simulink model "homeMobileManipulator"  (R2026a)
settings: Solver=ode4  StartTime=0  StopTime=Inf  FixedStep=cfg.rates.plant  MaxStep=cfg.rates.plant  AbsTol=1e-8
PostLoadFcn:
  | hmmSetup;
InitFcn:
  | hmmInitializeRun(bdroot);
values from neighbouring files (symbols this model uses):
  armJointLimits = zeros(numel(idx.arm), 2)    [hmmSetup.m]
  cfg = app.RunCfg    [HomeMobileManipulatorApp.m]    (also in HomeMobileManipulatorExample.m = params.cfg; hmmSetup.m = hmmConfig(); setupParams.m = data.cfg)
undefined symbols (not defined in the file or in its folder): actionQueueInit, actorNameTable, Angle, apertureMap, armPlanInit, Axis, basePlanInit, Custom, Extent, gray, gripperCoupling, invalidRayHits, movableRegistry, objectTargetInit, perceptionStatusInit, placeTargetInit, Position, robotStateInit, Sim3dSensor
libraries: robotmaniplib x20, robotcorelib x18, simulink x9, sim3dcameralib x6, sim3dgroundtruthsensorlib x4, dspmtrx3 x3, slpidlib x3, sim3dlib x3, hdlsllib x2, robotsim3dlib x1
(part 4 of 6)

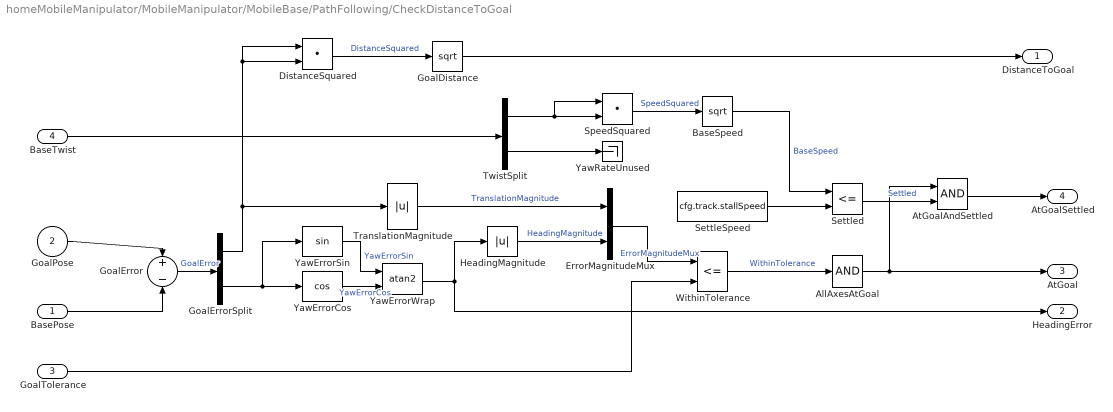
== system homeMobileManipulator/MobileManipulator/MobileBase/PathFollowing/CheckDistanceToGoal ==
  BasePose : Inport
  GoalPose : Inport  Port=2
  GoalTolerance : Inport  Port=3
  BaseTwist : Inport  Port=4
  AllAxesAtGoal : Logic  Inputs=1  IconShape=distinctive  AllPortsSameDT=off  OutDataTypeStr=boolean
  AtGoalAndSettled : Logic  Description=|  AllPortsSameDT=off  OutDataTypeStr=boolean
      | THE SUPERVISOR'S ARRIVAL TEST, WHICH IS NOT THE SAME SIGNAL THAT STOPS THE BASE.
      | 
      | AllAxesAtGoal alone is a POSITION test. Measured on the 40 s run of 2026-09-30 the
      | place leg reported HOLDING/DONE at t = 15.19 s while the chassis was still doing
      | 0.383 m/s, and the base then rolled a further 67.9 mm down its acceleration limit
      | (1.08 m/s^2, so 0.383^2/(2*1.08) = 67.9 mm - the ramp accounts for all of it). That is
      | more travel than the 80 mm per axis the goal was specified to, and it happens while the
      | arm is already planning: ArmSupervisor requested its place plan at 15.22 s, so the plan
      | was built on a base pose 64 mm stale.
      | 
      | cfg.track.goalHoldTime = 0.20 s does not catch this. It is a dwell on POSITION, and at
      | 0.4 m/s the chassis crosses 80 mm during the dwell, so the dwell is satisfied at cruise.
      | 
      | WHY THIS IS A SECOND SIGNAL AND NOT AN EXTRA TERM ON AtGoal. ZeroVelocityAtGoal in the
      | parent takes the RAW AllAxesAtGoal output and that is what commands zero velocity. AND
      | the settle term into that same signal and the command is never zeroed, so the base never
      | settles, so the term never becomes true - a deadlock. The raw test therefore stays on the
      | switch and only the signal leaving for BaseSupervisor carries the settle term. Because the
      | command is already zero by then, the plant decelerates at its own limit and this output is
      | guaranteed to go true within v/a, about 0.36 s on the measured run.
      | 
      | SAFE AGAINST THE STALL DETECTOR. BaseSupervisor/Following accumulates tProgress whenever
      | DistanceToGoal fails to improve by dProgressMin and declares Stalled at cfg.track.stallTime
      | = 2.00 s. Reconstructed from the same run, tProgress was 0.160 s at the arrival flip, so
      | there is 1.84 s of spare against the 0.36 s this adds.
      | 
      | TRANSLATION ONLY, DELIBERATELY. cfg.track.stallSpeed is in m/s. A yaw-rate term would need
      | a constant the configuration does not have, and the measured overshoot was pure translation
      | - vy and omega were both exactly zero from t = 15.08 s. Inventing a rate bound to cover a
      | case nothing has measured would be a worse trade than recording the limit here.
  BaseSpeed : Sqrt
  DistanceSquared : DotProduct  OutDataTypeStr=Inherit: Inherit via internal rule
  ErrorMagnitudeMux : Mux  Inputs=2
  GoalDistance : Sqrt
  GoalError : Sum  Inputs=+-
  GoalErrorSplit : Demux  Outputs=[2 1]
  HeadingMagnitude : Abs  SaturateOnIntegerOverflow=off
  SettleSpeed : Constant  Description=|  Value=cfg.track.stallSpeed
      | The speed below which the chassis counts as stopped. This is cfg.track.stallSpeed, the
      | same constant the stall detector already uses for "no progress", rather than a new one:
      | 0.020 m/s is either a speed worth noticing or it is not, and it cannot be both.
      | 
      | At this threshold the roll left after arrival is 0.020^2/(2*1.08) = 0.19 mm, against
      | 67.9 mm before the settle term existed.
  Settled : RelationalOperator  Operator=<=  OutDataTypeStr=boolean  RndMeth=Simplest  InputSameDT=off
  SpeedSquared : DotProduct  OutDataTypeStr=Inherit: Inherit via internal rule
  TranslationMagnitude : Abs  SaturateOnIntegerOverflow=off
  TwistSplit : Demux  Description=|  Outputs=[2 1]
      | BaseTwist is the REALISED body-frame [vx vy omega] after wheel saturation, not the
      | command - which is the whole point, since the command is already zero while the chassis
      | is still rolling. Split [2 1] so the translational pair can be normed on its own; the
      | yaw rate is deliberately not used, see AtGoalAndSettled.
  WithinTolerance : RelationalOperator  Operator=<=  OutDataTypeStr=boolean  RndMeth=Simplest  InputSameDT=off
  YawErrorCos : Trigonometry  Operator=cos
  YawErrorSin : Trigonometry
  YawErrorWrap : Trigonometry  Operator=atan2
  YawRateUnused : Terminator
  DistanceToGoal : Outport
  HeadingError : Outport  Port=2
  AtGoal : Outport  Port=3
  AtGoalSettled : Outport  Port=4
  wires:
  AtGoalAndSettled/1 -> AtGoalSettled/1
  Settled/1 -> AtGoalAndSettled/2  "Settled"
  SettleSpeed/1 -> Settled/2
  BaseSpeed/1 -> Settled/1  "BaseSpeed"
  GoalTolerance/1 -> WithinTolerance/2
  SpeedSquared/1 -> BaseSpeed/1  "SpeedSquared"
  HeadingMagnitude/1 -> ErrorMagnitudeMux/2  "HeadingMagnitude"
  TwistSplit/2 -> YawRateUnused/1
  YawErrorWrap/1 -> HeadingMagnitude/1, HeadingError/1
  AllAxesAtGoal/1 -> AtGoal/1, AtGoalAndSettled/1
  TranslationMagnitude/1 -> ErrorMagnitudeMux/1  "TranslationMagnitude"
  ErrorMagnitudeMux/1 -> WithinTolerance/1  "ErrorMagnitudeMux"
  BaseTwist/1 -> TwistSplit/1
  GoalDistance/1 -> DistanceToGoal/1
  DistanceSquared/1 -> GoalDistance/1  "DistanceSquared"
  WithinTolerance/1 -> AllAxesAtGoal/1  "WithinTolerance"
  YawErrorSin/1 -> YawErrorWrap/1  "YawErrorSin"
  GoalErrorSplit/2 -> YawErrorSin/1, YawErrorCos/1
  GoalErrorSplit/1 -> DistanceSquared/2, DistanceSquared/1, TranslationMagnitude/1
  GoalError/1 -> GoalErrorSplit/1  "GoalError"
  BasePose/1 -> GoalError/2
  GoalPose/1 -> GoalError/1
  TwistSplit/1 -> SpeedSquared/1, SpeedSquared/2
  YawErrorCos/1 -> YawErrorWrap/2  "YawErrorCos"

== system homeMobileManipulator/MobileManipulator/MobileBase/PathFollowing/ReferenceSample ==
  FollowTime : Inport
  Duration : Inport  Port=2
  RefTime : Inport  Port=3
  RefPose : Inport  Port=4
  RefVel : Inport  Port=5
  ClampTime : MinMax  Inputs=2
  RefAccelUnused : Terminator
  ReferenceTrajectory : robotcorelib/Polynomial Trajectory  Description=Robotics System Toolbox Polynomial Trajectory (cubic Hermite): the base reference at FollowTime, through the planner's timed samples with the planner's own velocities as boundary conditions. Replaces a hand-wired PreLookup + Direct Lookup Table linear blend (2026-10-08).  WaypointSource=External  Waypoints=[ 0, 2, 1, 5, 0; -1, 3, 1, 4, 4 ]  TimePoints=[ 0, 1, 2, 3, 4 ]  TimeInterval=[ 1, 4 ]  Method=Cubic Polynomial  ParameterSource=External  VelocityBoundaryCondition=zeros( 2, 5 )  AccelerationBoundaryCondition=zeros( 2, 5 )  SimulateUsing=Code generation
  RefPoseNow : Outport
  RefVelNow : Outport  Port=2
  wires:
  ReferenceTrajectory/3 -> RefAccelUnused/1
  RefTime/1 -> ReferenceTrajectory/3
  RefPose/1 -> ReferenceTrajectory/2
  ReferenceTrajectory/2 -> RefVelNow/1
  ClampTime/1 -> ReferenceTrajectory/1  "ClampTime"
  Duration/1 -> ClampTime/2
  ReferenceTrajectory/1 -> RefPoseNow/1
  FollowTime/1 -> ClampTime/1
  RefVel/1 -> ReferenceTrajectory/4

== system homeMobileManipulator/MobileManipulator/MobileBase/PathFollowing/TrackingError ==
  RefPoseNow : Inport
  RefVelNow : Inport  Port=2
  BasePose : Inport  Port=3
  BodyRotation : Subsystem
  CrossTrackMagnitude : Abs  SaturateOnIntegerOverflow=off
  ErrorBodySplit : Demux  Outputs=[1 1]
  ErrorSplit : Demux  Outputs=[2 1]
  ErrorToBody : Product  Multiplication=Matrix(*)
  FeedforwardMux : Mux  Inputs=2
  FeedforwardToBody : Product  Multiplication=Matrix(*)
  PoseErrorMux : Mux  Inputs=3
  PoseErrorWorld : Sum  Inputs=+-
  RefVelSplit : Demux  Outputs=[2 1]
  YawErrorCos : Trigonometry  Operator=cos
  YawErrorSin : Trigonometry
  YawErrorWrap : Trigonometry  Operator=atan2
  PoseErrorBody : Outport
  FeedforwardBody : Outport  Port=2
  CrossTrackError : Outport  Port=3
  wires:
  PoseErrorMux/1 -> PoseErrorBody/1  "PoseErrorMux"
  CrossTrackMagnitude/1 -> CrossTrackError/1
  ErrorBodySplit/2 -> CrossTrackMagnitude/1, PoseErrorMux/2
  ErrorBodySplit/1 -> PoseErrorMux/1
  FeedforwardMux/1 -> FeedforwardBody/1  "FeedforwardMux"
  YawErrorWrap/1 -> PoseErrorMux/3  "YawErrorWrap"
  YawErrorCos/1 -> YawErrorWrap/2  "YawErrorCos"
  YawErrorSin/1 -> YawErrorWrap/1  "YawErrorSin"
  FeedforwardToBody/1 -> FeedforwardMux/1  "FeedforwardToBody"
  ErrorSplit/2 -> YawErrorSin/1, YawErrorCos/1
  ErrorSplit/1 -> ErrorToBody/2
  RefVelSplit/1 -> FeedforwardToBody/2
  BodyRotation/1(RotBodyFromWorld) -> ErrorToBody/1, FeedforwardToBody/1
  RefVelSplit/2 -> FeedforwardMux/2
  PoseErrorWorld/1 -> ErrorSplit/1  "PoseErrorWorld"
  RefVelNow/1 -> RefVelSplit/1
  BasePose/1 -> BodyRotation/1(BasePose), PoseErrorWorld/2
  ErrorToBody/1 -> ErrorBodySplit/1  "ErrorToBody"
  RefPoseNow/1 -> PoseErrorWorld/1

== system homeMobileManipulator/MobileManipulator/Plant/BaseKinematics/PoseIntegration ==
  TwistRealised : Inport
  CosHeading : Trigonometry  Operator=cos
  HeadingIntegrator : Integrator  InitialCondition=cfg.base.initialPose(3)
  PoseAssemble : Mux  Inputs=2
  SinHeading : Trigonometry
  TwistSplit : Demux  Outputs=3
  VxCos : Product
  VxSin : Product
  VyCos : Product
  VySin : Product
  XDot : Sum  Inputs=+-
  XYIntegrator : Integrator  InitialCondition=cfg.base.initialPose(1:2)
  XYRate : Mux  Inputs=2
  YDot : Sum  Inputs=|++
  BasePose : Outport
  wires:
  PoseAssemble/1 -> BasePose/1  "BasePose"
  XYIntegrator/1 -> PoseAssemble/1  "XYWorld"
  XYRate/1 -> XYIntegrator/1
  YDot/1 -> XYRate/2  "YDotWorld"
  XDot/1 -> XYRate/1  "XDotWorld"
  VyCos/1 -> YDot/2  "VyCos"
  VxSin/1 -> YDot/1  "VxSin"
  VySin/1 -> XDot/2  "VySin"
  SinHeading/1 -> VySin/2, VxSin/2  "SinHeading"
  VxCos/1 -> XDot/1  "VxCos"
  CosHeading/1 -> VyCos/2, VxCos/2  "CosHeading"
  HeadingIntegrator/1 -> SinHeading/1, PoseAssemble/2, CosHeading/1  "Heading"
  TwistSplit/3 -> HeadingIntegrator/1  "OmegaBody"
  TwistSplit/2 -> VySin/1, VyCos/1  "VyBody"
  TwistRealised/1 -> TwistSplit/1
  TwistSplit/1 -> VxSin/1, VxCos/1  "VxBody"

== system homeMobileManipulator/MobileManipulator/Plant/BaseKinematics/WheelKinematics ==
  TwistCmd : Inport
  InverseWheel : Gain  Gain=cfg.base.wheelMatrix  Multiplication=Matrix(K*u)
  TwistLimit : Saturate  UpperLimit=[cfg.base.vxMax; cfg.base.vyMax; cfg.base.omegaMax]  LowerLimit=-[cfg.base.vxMax; cfg.base.vyMax; cfg.base.omegaMax]
  TwistRecovery : Gain  Gain=cfg.base.twistMatrix  Multiplication=Matrix(K*u)
  WheelLimit : Saturate  UpperLimit=cfg.base.wheelSpeedMax  LowerLimit=-cfg.base.wheelSpeedMax
  WheelSpeeds : Outport
  TwistRealised : Outport  Port=2
  wires:
  TwistRecovery/1 -> TwistRealised/1  "TwistRealised"
  WheelLimit/1 -> TwistRecovery/1, WheelSpeeds/1  "WheelSpeeds"
  InverseWheel/1 -> WheelLimit/1  "WheelSpeedsUnlimited"
  TwistLimit/1 -> InverseWheel/1  "TwistCmdLimited"
  TwistCmd/1 -> TwistLimit/1

== system homeMobileManipulator/MobileManipulator/Plant/CameraRig/Camera_1 ==
  CameraFrameBus : BusCreator  Inputs=11  OutDataTypeStr=Bus: CameraFrame  NonVirtualBus=on
      settings: InheritFromInputs=off
  CameraIndex : Constant  OutDataTypeStr=uint8
  CaptureTime : DigitalClock  SampleTime=cfg.rates.perception
  DepthRays : sim3dgroundtruthsensorlib/Simulation 3D Ray Tracer  Priority=1  sensorTag=Sim3dSensor�  sensorId=17  sensorName=Sim3dSensor�  vehTagList={'ApartmentShell';'Custom ...';'HomeMobileManipulator';'Scene Origin';'SceneProps'}  vehTag=ApartmentShell  CoordinateSystem=Default  mountLoc=Origin  offsetFlag=on  tmountOffset=cfg.camera.fixed(1).translation  rmountOffset=cfg.camera.fixed(1).rotation  RayOrigins=rays.origins  RayDirections=rays.directions  RayLengths=rays.lengths  NumberOfBounces=cfg.depth.rayBounces  VisualizeTraceLines=off  EnableOptimization=on  SampleTime=cfg.rates.perception  mountPoint=[0.5 -2.5 2.3]  mountOrientation=[0 -0.698131700797732 0.197395559849881]  aMode=5  ID=17
      settings: LibrarySourceBlock=sl3dlib/Simulation 3D/Sensors/Simulation 3D Ray Tracer
  DepthSourceRayTrace : Constant  Value=cfg.depth.SOURCE_RAYTRACE  OutDataTypeStr=uint8
  FixedCam : sim3dcameralib/Simulation 3D Camera  Priority=1  sensorTag=Sim3dSensor�  sensorId=18  sensorName=Sim3dSensor�  vehTagList={'ApartmentShell';'Custom ...';'HomeMobileManipulator';'Scene Origin';'SceneProps'}  vehTag=ApartmentShell  CoordinateSystem=Default  mountLoc=Origin  offsetFlag=on  tmountOffset=cfg.camera.fixed(1).translation  extTmount=off  rmountOffset=cfg.camera.fixed(1).rotation  extRmount=off  FocalLength=cfg.camera.focalLength  OpticalCenter=cfg.camera.opticalCenter  ImageSize=cfg.camera.imageSize  RadialDistortion=[0, 0]  TangentialDistortion=[0, 0]  SensorSkew=0  VisualizeFieldOfView=off  FieldOfViewRange=61  DepthOutportEnabled=on  SemanticOutportEnabled=off  TransformOutportEnabled=on  SampleTime=cfg.rates.perception  mountPoint=[0.5 -2.5 2.3]  mountOrientation=[0 -0.698131700797732 0.197395559849881]  aMode=aMode  ID=18
  FrameValid : Constant  OutDataTypeStr=boolean
  HitNormalsUnused : Terminator
  ImageSizePx : Constant  Value=cfg.camera.imageSize(:)  OutDataTypeStr=uint16
  Intrinsics : Constant  Value=[cfg.camera.focalLength(:); cfg.camera.opticalCenter(:)]
  RayGridSize : Constant  Value=cfg.depth.rayGrid(:)  OutDataTypeStr=uint16
  RayHitsBus : BusCreator  Inputs=5  OutDataTypeStr=Bus: RayHits  NonVirtualBus=on
      settings: InheritFromInputs=off
  CameraFrame : Outport  OutDataTypeStr=Bus: CameraFrame  BusOutputAsStruct=on
  wires:
  CameraFrameBus/1 -> CameraFrame/1
  CaptureTime/1 -> CameraFrameBus/10
  FrameValid/1 -> CameraFrameBus/11
  ImageSizePx/1 -> CameraFrameBus/7
  Intrinsics/1 -> CameraFrameBus/6
  FixedCam/3 -> CameraFrameBus/8
  FixedCam/2 -> CameraFrameBus/3
  FixedCam/1 -> CameraFrameBus/2
  RayHitsBus/1 -> CameraFrameBus/5
  CameraIndex/1 -> CameraFrameBus/1
  FixedCam/4 -> CameraFrameBus/9
  RayGridSize/1 -> RayHitsBus/5
  DepthSourceRayTrace/1 -> CameraFrameBus/4
  DepthRays/5 -> RayHitsBus/2
  DepthRays/4 -> RayHitsBus/4
  DepthRays/3 -> RayHitsBus/1
  DepthRays/2 -> HitNormalsUnused/1
  DepthRays/1 -> RayHitsBus/3

== system homeMobileManipulator/MobileManipulator/Plant/CameraRig/Camera_2 ==
  CameraFrameBus : BusCreator  Inputs=11  OutDataTypeStr=Bus: CameraFrame  NonVirtualBus=on
      settings: InheritFromInputs=off
  CameraIndex : Constant  Value=2  OutDataTypeStr=uint8
  CaptureTime : DigitalClock  SampleTime=cfg.rates.perception
  DepthRays : sim3dgroundtruthsensorlib/Simulation 3D Ray Tracer  Priority=1  sensorTag=Sim3dSensor�  sensorId=19  sensorName=Sim3dSensor�  vehTagList={'ApartmentShell';'Custom ...';'HomeMobileManipulator';'Scene Origin';'SceneProps'}  vehTag=ApartmentShell  CoordinateSystem=Default  mountLoc=Origin  offsetFlag=on  tmountOffset=cfg.camera.fixed(2).translation  rmountOffset=cfg.camera.fixed(2).rotation  RayOrigins=rays.origins  RayDirections=rays.directions  RayLengths=rays.lengths  NumberOfBounces=cfg.depth.rayBounces  VisualizeTraceLines=off  EnableOptimization=on  SampleTime=cfg.rates.perception  mountPoint=[4 -5.6 2.3]  mountOrientation=[0 -0.698131700797732 -2.40877755180329]  aMode=5  ID=19
      settings: LibrarySourceBlock=sl3dlib/Simulation 3D/Sensors/Simulation 3D Ray Tracer
  DepthSourceRayTrace : Constant  Value=cfg.depth.SOURCE_RAYTRACE  OutDataTypeStr=uint8
  FixedCam : sim3dcameralib/Simulation 3D Camera  Priority=1  sensorTag=Sim3dSensor�  sensorId=20  sensorName=Sim3dSensor�  vehTagList={'ApartmentShell';'Custom ...';'HomeMobileManipulator';'Scene Origin';'SceneProps'}  vehTag=ApartmentShell  CoordinateSystem=Default  mountLoc=Origin  offsetFlag=on  tmountOffset=cfg.camera.fixed(2).translation  extTmount=off  rmountOffset=cfg.camera.fixed(2).rotation  extRmount=off  FocalLength=cfg.camera.focalLength  OpticalCenter=cfg.camera.opticalCenter  ImageSize=cfg.camera.imageSize  RadialDistortion=[0, 0]  TangentialDistortion=[0, 0]  SensorSkew=0  VisualizeFieldOfView=off  FieldOfViewRange=61  DepthOutportEnabled=on  SemanticOutportEnabled=off  TransformOutportEnabled=on  SampleTime=cfg.rates.perception  mountPoint=[4 -5.6 2.3]  mountOrientation=[0 -0.698131700797732 -2.40877755180329]  aMode=aMode  ID=20
  FrameValid : Constant  OutDataTypeStr=boolean
  HitNormalsUnused : Terminator
  ImageSizePx : Constant  Value=cfg.camera.imageSize(:)  OutDataTypeStr=uint16
  Intrinsics : Constant  Value=[cfg.camera.focalLength(:); cfg.camera.opticalCenter(:)]
  RayGridSize : Constant  Value=cfg.depth.rayGrid(:)  OutDataTypeStr=uint16
  RayHitsBus : BusCreator  Inputs=5  OutDataTypeStr=Bus: RayHits  NonVirtualBus=on
      settings: InheritFromInputs=off
  CameraFrame : Outport  OutDataTypeStr=Bus: CameraFrame  BusOutputAsStruct=on
  wires:
  CameraFrameBus/1 -> CameraFrame/1
  FrameValid/1 -> CameraFrameBus/11
  CaptureTime/1 -> CameraFrameBus/10
  Intrinsics/1 -> CameraFrameBus/6
  FixedCam/3 -> CameraFrameBus/8
  FixedCam/4 -> CameraFrameBus/9
  FixedCam/1 -> CameraFrameBus/2
  FixedCam/2 -> CameraFrameBus/3
  ImageSizePx/1 -> CameraFrameBus/7
  RayHitsBus/1 -> CameraFrameBus/5
  DepthSourceRayTrace/1 -> CameraFrameBus/4
  CameraIndex/1 -> CameraFrameBus/1
  DepthRays/5 -> RayHitsBus/2
  RayGridSize/1 -> RayHitsBus/5
  DepthRays/4 -> RayHitsBus/4
  DepthRays/3 -> RayHitsBus/1
  DepthRays/2 -> HitNormalsUnused/1
  DepthRays/1 -> RayHitsBus/3

== system homeMobileManipulator/MobileManipulator/Plant/CameraRig/Camera_3 ==
  CameraFrameBus : BusCreator  Inputs=11  OutDataTypeStr=Bus: CameraFrame  NonVirtualBus=on
      settings: InheritFromInputs=off
  CameraIndex : Constant  Value=3  OutDataTypeStr=uint8
  CaptureTime : DigitalClock  SampleTime=cfg.rates.perception
  DepthRays : sim3dgroundtruthsensorlib/Simulation 3D Ray Tracer  Priority=1  sensorTag=Sim3dSensor�  sensorId=21  sensorName=Sim3dSensor�  vehTagList={'ApartmentShell';'Custom ...';'HomeMobileManipulator';'Scene Origin';'SceneProps'}  vehTag=ApartmentShell  CoordinateSystem=Default  mountLoc=Origin  offsetFlag=on  tmountOffset=cfg.camera.fixed(3).translation  rmountOffset=cfg.camera.fixed(3).rotation  RayOrigins=rays.origins  RayDirections=rays.directions  RayLengths=rays.lengths  NumberOfBounces=cfg.depth.rayBounces  VisualizeTraceLines=off  EnableOptimization=on  SampleTime=cfg.rates.perception  mountPoint=[6.5 -4.5 2.3]  mountOrientation=[0 -0.698131700797732 -0.588002603547568]  aMode=5  ID=21
      settings: LibrarySourceBlock=sl3dlib/Simulation 3D/Sensors/Simulation 3D Ray Tracer
  DepthSourceRayTrace : Constant  Value=cfg.depth.SOURCE_RAYTRACE  OutDataTypeStr=uint8
  FixedCam : sim3dcameralib/Simulation 3D Camera  Priority=1  sensorTag=Sim3dSensor�  sensorId=22  sensorName=Sim3dSensor�  vehTagList={'ApartmentShell';'Custom ...';'HomeMobileManipulator';'Scene Origin';'SceneProps'}  vehTag=ApartmentShell  CoordinateSystem=Default  mountLoc=Origin  offsetFlag=on  tmountOffset=cfg.camera.fixed(3).translation  extTmount=off  rmountOffset=cfg.camera.fixed(3).rotation  extRmount=off  FocalLength=cfg.camera.focalLength  OpticalCenter=cfg.camera.opticalCenter  ImageSize=cfg.camera.imageSize  RadialDistortion=[0, 0]  TangentialDistortion=[0, 0]  SensorSkew=0  VisualizeFieldOfView=off  FieldOfViewRange=61  DepthOutportEnabled=on  SemanticOutportEnabled=off  TransformOutportEnabled=on  SampleTime=cfg.rates.perception  mountPoint=[6.5 -4.5 2.3]  mountOrientation=[0 -0.698131700797732 -0.588002603547568]  aMode=aMode  ID=22
  FrameValid : Constant  OutDataTypeStr=boolean
  HitNormalsUnused : Terminator
  ImageSizePx : Constant  Value=cfg.camera.imageSize(:)  OutDataTypeStr=uint16
  Intrinsics : Constant  Value=[cfg.camera.focalLength(:); cfg.camera.opticalCenter(:)]
  RayGridSize : Constant  Value=cfg.depth.rayGrid(:)  OutDataTypeStr=uint16
  RayHitsBus : BusCreator  Inputs=5  OutDataTypeStr=Bus: RayHits  NonVirtualBus=on
      settings: InheritFromInputs=off
  CameraFrame : Outport  OutDataTypeStr=Bus: CameraFrame  BusOutputAsStruct=on
  wires:
  CameraFrameBus/1 -> CameraFrame/1
  FrameValid/1 -> CameraFrameBus/11
  ImageSizePx/1 -> CameraFrameBus/7
  Intrinsics/1 -> CameraFrameBus/6
  FixedCam/4 -> CameraFrameBus/9
  FixedCam/2 -> CameraFrameBus/3
  FixedCam/3 -> CameraFrameBus/8
  RayHitsBus/1 -> CameraFrameBus/5
  CameraIndex/1 -> CameraFrameBus/1
  RayGridSize/1 -> RayHitsBus/5
  DepthSourceRayTrace/1 -> CameraFrameBus/4
  CaptureTime/1 -> CameraFrameBus/10
  DepthRays/5 -> RayHitsBus/2
  DepthRays/4 -> RayHitsBus/4
  DepthRays/3 -> RayHitsBus/1
  DepthRays/2 -> HitNormalsUnused/1
  DepthRays/1 -> RayHitsBus/3
  FixedCam/1 -> CameraFrameBus/2

== system homeMobileManipulator/MobileManipulator/Plant/CameraRig/Camera_4 ==
  CameraFrameBus : BusCreator  Inputs=11  OutDataTypeStr=Bus: CameraFrame  NonVirtualBus=on
      settings: InheritFromInputs=off
  CameraIndex : Constant  Value=4  OutDataTypeStr=uint8
  CaptureTime : DigitalClock  SampleTime=cfg.rates.perception
  DepthRays : sim3dgroundtruthsensorlib/Simulation 3D Ray Tracer  Priority=1  sensorTag=Sim3dSensor�  sensorId=23  sensorName=Sim3dSensor�  vehTagList={'ApartmentShell';'Custom ...';'HomeMobileManipulator';'Scene Origin';'SceneProps'}  vehTag=ApartmentShell  CoordinateSystem=Default  mountLoc=Origin  offsetFlag=on  tmountOffset=cfg.camera.fixed(4).translation  rmountOffset=cfg.camera.fixed(4).rotation  RayOrigins=rays.origins  RayDirections=rays.directions  RayLengths=rays.lengths  NumberOfBounces=cfg.depth.rayBounces  VisualizeTraceLines=off  EnableOptimization=on  SampleTime=cfg.rates.perception  mountPoint=[6.5 -2.5 2.3]  mountOrientation=[0 -0.698131700797732 0.588002603547568]  aMode=5  ID=23
      settings: LibrarySourceBlock=sl3dlib/Simulation 3D/Sensors/Simulation 3D Ray Tracer
  DepthSourceRayTrace : Constant  Value=cfg.depth.SOURCE_RAYTRACE  OutDataTypeStr=uint8
  FixedCam : sim3dcameralib/Simulation 3D Camera  Priority=1  sensorTag=Sim3dSensor�  sensorId=24  sensorName=Sim3dSensor�  vehTagList={'ApartmentShell';'Custom ...';'HomeMobileManipulator';'Scene Origin';'SceneProps'}  vehTag=ApartmentShell  CoordinateSystem=Default  mountLoc=Origin  offsetFlag=on  tmountOffset=cfg.camera.fixed(4).translation  extTmount=off  rmountOffset=cfg.camera.fixed(4).rotation  extRmount=off  FocalLength=cfg.camera.focalLength  OpticalCenter=cfg.camera.opticalCenter  ImageSize=cfg.camera.imageSize  RadialDistortion=[0, 0]  TangentialDistortion=[0, 0]  SensorSkew=0  VisualizeFieldOfView=off  FieldOfViewRange=61  DepthOutportEnabled=on  SemanticOutportEnabled=off  TransformOutportEnabled=on  SampleTime=cfg.rates.perception  mountPoint=[6.5 -2.5 2.3]  mountOrientation=[0 -0.698131700797732 0.588002603547568]  aMode=aMode  ID=24
  FrameValid : Constant  OutDataTypeStr=boolean
  HitNormalsUnused : Terminator
  ImageSizePx : Constant  Value=cfg.camera.imageSize(:)  OutDataTypeStr=uint16
  Intrinsics : Constant  Value=[cfg.camera.focalLength(:); cfg.camera.opticalCenter(:)]
  RayGridSize : Constant  Value=cfg.depth.rayGrid(:)  OutDataTypeStr=uint16
  RayHitsBus : BusCreator  Inputs=5  OutDataTypeStr=Bus: RayHits  NonVirtualBus=on
      settings: InheritFromInputs=off
  CameraFrame : Outport  OutDataTypeStr=Bus: CameraFrame  BusOutputAsStruct=on
  wires:
  FrameValid/1 -> CameraFrameBus/11
  CaptureTime/1 -> CameraFrameBus/10
  ImageSizePx/1 -> CameraFrameBus/7
  Intrinsics/1 -> CameraFrameBus/6
  FixedCam/3 -> CameraFrameBus/8
  FixedCam/4 -> CameraFrameBus/9
  CameraFrameBus/1 -> CameraFrame/1
  FixedCam/1 -> CameraFrameBus/2
  FixedCam/2 -> CameraFrameBus/3
  RayHitsBus/1 -> CameraFrameBus/5
  DepthSourceRayTrace/1 -> CameraFrameBus/4
  RayGridSize/1 -> RayHitsBus/5
  CameraIndex/1 -> CameraFrameBus/1
  DepthRays/5 -> RayHitsBus/2
  DepthRays/4 -> RayHitsBus/4
  DepthRays/3 -> RayHitsBus/1
  DepthRays/2 -> HitNormalsUnused/1
  DepthRays/1 -> RayHitsBus/3

== system homeMobileManipulator/MobileManipulator/Plant/CameraRig/WristCamera ==
  RobotConfig : Inport
  CalibInvalid : BusCreator  Inputs=5  OutDataTypeStr=Bus: RayHits  NonVirtualBus=on
      settings: InheritFromInputs=off
  CameraFrameBus : BusCreator  Inputs=11  OutDataTypeStr=Bus: CameraFrame  NonVirtualBus=on
      settings: InheritFromInputs=off
  CameraIndex : Constant  Value=cfg.camera.wrist.index  OutDataTypeStr=uint8  SampleTime=cfg.rates.perception
  CaptureTime : DigitalClock  SampleTime=cfg.rates.perception
  DepthSourceRender : Constant  Value=cfg.depth.SOURCE_RENDER  OutDataTypeStr=uint8  SampleTime=cfg.rates.perception
  FrameValid : Constant  OutDataTypeStr=boolean  SampleTime=cfg.rates.perception
  GridSizeInvalid : Constant  Value=invalidRayHits.GridSize  OutDataTypeStr=uint16  SampleTime=cfg.rates.perception
  HitDistancesInvalid : Constant  Value=invalidRayHits.HitDistances  OutDataTypeStr=single  SampleTime=cfg.rates.perception
  HitLocationsInvalid : Constant  Value=invalidRayHits.HitLocations  OutDataTypeStr=single  SampleTime=cfg.rates.perception
  ImageSizePx : Constant  Value=cfg.camera.wrist.imageSize(:)  OutDataTypeStr=uint16  SampleTime=cfg.rates.perception
  Intrinsics : Constant  Value=[cfg.camera.wrist.focalLength(:); cfg.camera.wrist.opticalCenter(:)]  SampleTime=cfg.rates.perception
  IsValidHitInvalid : Constant  Value=invalidRayHits.IsValidHit  OutDataTypeStr=boolean  SampleTime=cfg.rates.perception
  SurfaceIdsInvalid : Constant  Value=invalidRayHits.SurfaceIds  OutDataTypeStr=uint32  SampleTime=cfg.rates.perception
  WristCam : sim3dcameralib/Simulation 3D Camera  Priority=1  sensorTag=Sim3dSensor�  sensorId=25  sensorName=Sim3dSensor�  vehTagList={'ApartmentShell';'Custom ...';'HomeMobileManipulator';'Scene Origin';'SceneProps'}  vehTag=Custom ...  parentTag=HomeMobileManipulator  CoordinateSystem=Default  mountLoc=Origin  offsetFlag=on  tmountOffset=[0, 0, 0]  extTmount=on  rmountOffset=[0, 0, 0]  extRmount=on  FocalLength=cfg.camera.wrist.focalLength  OpticalCenter=cfg.camera.wrist.opticalCenter  ImageSize=cfg.camera.wrist.imageSize  RadialDistortion=[0, 0]  TangentialDistortion=[0, 0]  SensorSkew=0  VisualizeFieldOfView=off  FieldOfViewRange=61  DepthOutportEnabled=on  SemanticOutportEnabled=off  TransformOutportEnabled=on  SampleTime=cfg.rates.perception  mountPoint=[0 0 0]  mountOrientation=[0 0 0]  aMode=aMode  ID=25
  WristMountPose : Subsystem
  CameraFrame : Outport  OutDataTypeStr=Bus: CameraFrame  BusOutputAsStruct=on
  wires:
  CameraFrameBus/1 -> CameraFrame/1
  FrameValid/1 -> CameraFrameBus/11
  CaptureTime/1 -> CameraFrameBus/10
  ImageSizePx/1 -> CameraFrameBus/7
  Intrinsics/1 -> CameraFrameBus/6
  WristCam/4 -> CameraFrameBus/9
  WristCam/2 -> CameraFrameBus/3
  WristCam/1 -> CameraFrameBus/2
  CalibInvalid/1 -> CameraFrameBus/5  "Calib"
  DepthSourceRender/1 -> CameraFrameBus/4
  CameraIndex/1 -> CameraFrameBus/1
  WristMountPose/2(RelRotation) -> WristCam/2  "RelRotation"
  WristMountPose/1(RelTranslation) -> WristCam/1  "RelTranslation"
  SurfaceIdsInvalid/1 -> CalibInvalid/4
  GridSizeInvalid/1 -> CalibInvalid/5
  HitLocationsInvalid/1 -> CalibInvalid/3
  IsValidHitInvalid/1 -> CalibInvalid/2
  HitDistancesInvalid/1 -> CalibInvalid/1
  RobotConfig/1 -> WristMountPose/1(RobotConfig)
  WristCam/3 -> CameraFrameBus/8

== system homeMobileManipulator/MobileManipulator/Plant/GraspCaptureGate/ActorNameLookup ==
  ActorId : Inport
  ActorNameTable : Constant  Value=actorNameTable
  IdToIndex : DataTypeConversion  Description=uint8 -> double before the clamp, because Saturation's limits are read in the input's own type: on a uint8 signal an upper limit of 20 is fine but the arithmetic that follows is modular, and an index is not a count of something that can wrap.  OutDataTypeStr=double
  NameRow : Selector  NumberOfDimensions=2  IndexOptions=Index vector (port),Select all  Indices=,1  OutputSizes=1,1
  RowClamp : Saturate  Description=|  UpperLimit=size(actorNameTable, 1)  LowerLimit=1
      | ActorId 0 IS THE "NO CANDIDATE" SENTINEL AND THERE IS NO ROW 0.
      | 
      | The clamp is to row 1 rather than to a sentinel name because Simulation 3D Robot dereferences the name BEFORE it consults ActivateGrasp - world.Actors.(name) is evaluated unconditionally - so the row has to name an actor that exists even when nothing is being grasped. Nothing attaches: with ActivateGrasp false, TargetGraspUtils takes its detach branch whichever valid actor is named.
      | 
      | The upper limit is size(actorNameTable, 1) rather than a number, so a longer prop manifest cannot make the index run off the end of the table.
  ActorName : Outport
  wires:
  NameRow/1 -> ActorName/1
  ActorNameTable/1 -> NameRow/1
  RowClamp/1 -> NameRow/2  "ClampedRow"
  IdToIndex/1 -> RowClamp/1  "RowIndex"
  ActorId/1 -> IdToIndex/1

== system homeMobileManipulator/MobileManipulator/Plant/GraspCaptureGate/ExtentMatch ==
  AchievedAperture : Inport
  CandidateExtent : Inport  Port=2
  AbsExtentError : Abs
  ExtentError : Sum  Inputs=+-
  ExtentMatchTol : Constant  Value=cfg.grasp.extentMatchTol
  ExtentMatched : RelationalOperator  Operator=<=  OutDataTypeStr=boolean  InputSameDT=off
  Match : Outport
  wires:
  ExtentMatchTol/1 -> ExtentMatched/2
  AbsExtentError/1 -> ExtentMatched/1  "AbsExtentError"
  ExtentMatched/1 -> Match/1
  ExtentError/1 -> AbsExtentError/1  "ExtentError"
  CandidateExtent/1 -> ExtentError/2
  AchievedAperture/1 -> ExtentError/1

== system homeMobileManipulator/MobileManipulator/Plant/GraspCaptureGate/GraspHold ==
  GraspRequest : Inport
  CaptureAuthorised : Inport  Port=2
  CaptureOrHolding : Logic  Operator=OR  IconShape=distinctive
  HeldPrev : UnitDelay  SampleTime=-1
  HoldWhileRequested : Logic  IconShape=distinctive
  Holding : Outport
  wires:
  HeldPrev/1 -> CaptureOrHolding/2
  CaptureAuthorised/1 -> CaptureOrHolding/1
  HoldWhileRequested/1 -> Holding/1, HeldPrev/1
  GraspRequest/1 -> HoldWhileRequested/1
  CaptureOrHolding/1 -> HoldWhileRequested/2  "CaptureOrHolding"

== system homeMobileManipulator/MobileManipulator/Plant/GraspCaptureGate/WithinCapture ==
  GraspFramePos : Inport
  CandidatePosition : Inport  Port=2
  NumInCapture : Inport  Port=3
  CaptureDistance : Sqrt
  CaptureGeometryOk : Logic  IconShape=distinctive  AllPortsSameDT=off  OutDataTypeStr=boolean
  CaptureRadius : Constant  Value=cfg.grasp.captureRadius
  Displacement : Sum  Inputs=+-
  ExactlyOneInCapture : RelationalOperator  Operator===  OutDataTypeStr=boolean  InputSameDT=off
  SingleCandidate : Constant  OutDataTypeStr=uint8
  SquaredDistance : DotProduct  OutDataTypeStr=Inherit: Inherit via internal rule
  WithinRadius : RelationalOperator  Operator=<=  OutDataTypeStr=boolean  InputSameDT=off
  InCapture : Outport
  wires:
  CaptureGeometryOk/1 -> InCapture/1
  ExactlyOneInCapture/1 -> CaptureGeometryOk/2  "ExactlyOneInCapture"
  WithinRadius/1 -> CaptureGeometryOk/1  "WithinRadius"
  SingleCandidate/1 -> ExactlyOneInCapture/2
  CaptureRadius/1 -> WithinRadius/2
  CaptureDistance/1 -> WithinRadius/1  "CaptureDistance"
  SquaredDistance/1 -> CaptureDistance/1  "SquaredRange"
  NumInCapture/1 -> ExactlyOneInCapture/1
  Displacement/1 -> SquaredDistance/1, SquaredDistance/2  "GraspOffset"
  CandidatePosition/1 -> Displacement/2
  GraspFramePos/1 -> Displacement/1

== system homeMobileManipulator/MobileManipulator/SafetyMonitor/StalenessCheck/ArmStale ==
  Now : Inport
  Timestamp : Inport  Port=2
  Timeout : Inport  Port=3
  Fresh : Inport  Port=4
  Age : Sum  Inputs=+-
  Expired : RelationalOperator  Operator=>
  StaleAndExpected : Logic  IconShape=distinctive
  Stale : Outport
  wires:
  Expired/1 -> StaleAndExpected/1  "Expired"
  Timeout/1 -> Expired/2
  Age/1 -> Expired/1  "Age"
  StaleAndExpected/1 -> Stale/1
  Timestamp/1 -> Age/2
  Now/1 -> Age/1
  Fresh/1 -> StaleAndExpected/2

== system homeMobileManipulator/MobileManipulator/SafetyMonitor/StalenessCheck/BaseStale ==
  Now : Inport
  Timestamp : Inport  Port=2
  Timeout : Inport  Port=3
  Fresh : Inport  Port=4
  Age : Sum  Inputs=+-
  Expired : RelationalOperator  Operator=>
  StaleAndExpected : Logic  IconShape=distinctive
  Stale : Outport
  wires:
  Expired/1 -> StaleAndExpected/1  "Expired"
  Fresh/1 -> StaleAndExpected/2
  Timeout/1 -> Expired/2
  StaleAndExpected/1 -> Stale/1
  Age/1 -> Expired/1  "Age"
  Timestamp/1 -> Age/2
  Now/1 -> Age/1

== system homeMobileManipulator/MobileManipulator/SafetyMonitor/StalenessCheck/ProviderStale ==
  Now : Inport
  Timestamp : Inport  Port=2
  Timeout : Inport  Port=3
  Fresh : Inport  Port=4
  Age : Sum  Inputs=+-
  Expired : RelationalOperator  Operator=>
  StaleAndExpected : Logic  IconShape=distinctive
  Stale : Outport
  wires:
  Fresh/1 -> StaleAndExpected/2
  Expired/1 -> StaleAndExpected/1  "Expired"
  Timeout/1 -> Expired/2
  Timestamp/1 -> Age/2
  StaleAndExpected/1 -> Stale/1
  Now/1 -> Age/1
  Age/1 -> Expired/1  "Age"

== system homeMobileManipulator/MobileManipulator/SafetyMonitor/StalenessCheck/StateStale ==
  Now : Inport
  Timestamp : Inport  Port=2
  Timeout : Inport  Port=3
  Fresh : Inport  Port=4
  Age : Sum  Inputs=+-
  Expired : RelationalOperator  Operator=>
  StaleAndExpected : Logic  IconShape=distinctive
  Stale : Outport
  wires:
  StaleAndExpected/1 -> Stale/1
  Expired/1 -> StaleAndExpected/1  "Expired"
  Fresh/1 -> StaleAndExpected/2
  Timeout/1 -> Expired/2
  Age/1 -> Expired/1  "Age"
  Timestamp/1 -> Age/2
  Now/1 -> Age/1

== system homeMobileManipulator/MobileManipulator/SafetyMonitor/WorkspaceCheck/ToolPoseInArmFrame ==
  ArmConfig : Inport
  ConfigRow : Math  Operator=transpose
  FullConfig : Mux  Inputs=2
  GripperZero : Constant  Value=zeros(cfg.gripper.nJoints, 1)
  ToolTransform : robotmaniplib/Get Transform  RigidBodyTree=armIkTree  SourceBody=tcp_frame  TargetBody=arm_mount  SimulateUsing=Code generation
  TranslationHomogeneous : Product  Multiplication=Matrix(*)
  TranslationPick : Constant  Value=[0;0;0;1]
  TranslationSelect : Gain  Gain=[eye(3), zeros(3,1)]  Multiplication=Matrix(K*u)
  ToolTranslation : Outport
  wires:
  TranslationSelect/1 -> ToolTranslation/1  "TranslationSelect"
  ToolTransform/1 -> TranslationHomogeneous/1
  FullConfig/1 -> ConfigRow/1  "FullConfig"
  TranslationPick/1 -> TranslationHomogeneous/2
  TranslationHomogeneous/1 -> TranslationSelect/1  "TranslationHomogeneous"
  GripperZero/1 -> FullConfig/2
  ConfigRow/1 -> ToolTransform/1  "ConfigRow"
  ArmConfig/1 -> FullConfig/1

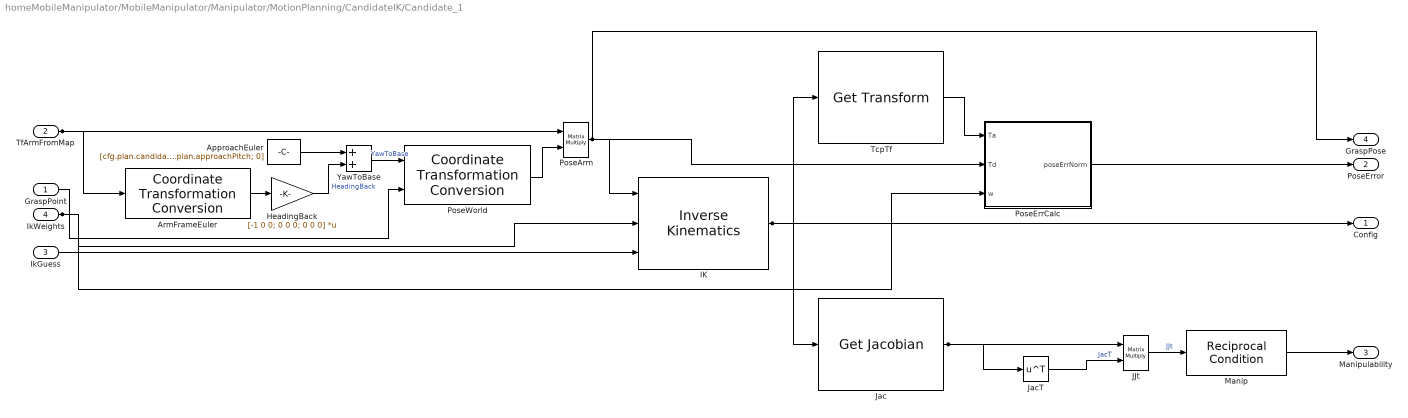
== system homeMobileManipulator/MobileManipulator/Manipulator/MotionPlanning/CandidateIK/Candidate_1 ==
  GraspPoint : Inport
  TfArmFromMap : Inport  Port=2
  IkGuess : Inport  Port=3
  IkWeights : Inport  Port=4
  ApproachEuler : Constant  Value=[cfg.plan.candidateYaw(1); cfg.plan.approachPitch; 0]
  ArmFrameEuler : robotcorelib/Coordinate Transformation Conversion  InputRepresentation=Homogeneous Transformation  InputEulerSequence=ZYX  ShowTrVecInputPort=off  OutputRepresentation=Euler Angles  OutputEulerSequence=ZYX  ShowTrVecOutputPort=off  SimulateUsing=Code generation
  HeadingBack : Gain  Gain=[-1 0 0; 0 0 0; 0 0 0]  Multiplication=Matrix(K*u)
  IK : robotmaniplib/Inverse Kinematics  RigidBodyTree=armIkTree  EndEffector=tcp_frame  ShowInfo=off  SolverName=BFGS Gradient Projection  EnforceJointLimits=on  AllowRandomRestarts=on  MaxIterations=cfg.plan.ikMaxIterations  MaxTime=cfg.plan.ikMaxTime  GradientTolerance=1e-7  SolutionTolerance=1e-6  StepTolerance=1e-14  ConstraintTolerance=1e-6  ErrorChangeTolerance=1e-12  UseErrorDamping=on  DampingBias=0.0025  RandomStream=mt19937ar with seed  Seed=cfg.plan.ikSeed  SimulateUsing=Code generation
  JJt : Product  Multiplication=Matrix(*)
  Jac : robotmaniplib/Get Jacobian  RigidBodyTree=armIkTree  EndEffector=tcp_frame  SimulateUsing=Code generation
  JacT : Math  Operator=transpose  SignedPower=on  RndMeth=Zero
  Manip : dspmtrx3/Reciprocal Condition
  PoseArm : Product  Multiplication=Matrix(*)
  PoseErrCalc : Subsystem  Description=Weighted twist between the achieved (Ta) and desired (Td) tool pose - the Inverse Kinematics block's PoseErrorNorm, rebuilt because its Info port cannot compile in this release. Blocks replace the former MATLAB Function (2026-10-14): inv(Ta)*Td, Coordinate Transformation Conversion to axis-angle and translation, weights in RST order (3 orientation, 3 position), 2-norm. Matched the function to 6.3e-9 worst case over 300 pose pairs, 2e-17 median.
  PoseWorld : robotcorelib/Coordinate Transformation Conversion  InputRepresentation=Euler Angles  InputEulerSequence=ZYX  ShowTrVecInputPort=on  OutputRepresentation=Homogeneous Transformation  OutputEulerSequence=ZYX  ShowTrVecOutputPort=off  SimulateUsing=Code generation
  TcpTf : robotmaniplib/Get Transform  RigidBodyTree=armIkTree  SourceBody=tcp_frame  TargetBody=arm_mount  SimulateUsing=Code generation
  YawToBase : Sum  Description=Re-express the map-frame ZYX Euler triple so its yaw is measured from the ARM base. PoseArm = TfArmFromMap * PoseWorld would otherwise reduce the yaw by the base heading, aiming the jaws (and the wrist camera) relative to the room; adding the heading back makes cfg.plan.candidateYaw mean yaw about the arm base vertical. TfArmFromMap's rotation is Rz(-heading), so ArmFrameEuler's first element is -heading and HeadingBack flips its sign. Replaces a MATLAB Function (heading = -atan2(T21,T11)) with Robotics System Toolbox blocks.
  Config : Outport
  PoseError : Outport  Port=2
  Manipulability : Outport  Port=3
  GraspPose : Outport  Port=4
  wires:
  Manip/1 -> Manipulability/1
  JJt/1 -> Manip/1  "JJt"
  JacT/1 -> JJt/2  "JacT"
  PoseErrCalc/1(poseErrNorm) -> PoseError/1
  Jac/1 -> JacT/1, JJt/1
  TcpTf/1 -> PoseErrCalc/1(Ta)
  IK/1 -> Config/1, Jac/1, TcpTf/1
  IkGuess/1 -> IK/3
  IkWeights/1 -> PoseErrCalc/3(w), IK/2
  ApproachEuler/1 -> YawToBase/1
  PoseWorld/1 -> PoseArm/2
  GraspPoint/1 -> PoseWorld/2
  ArmFrameEuler/1 -> HeadingBack/1
  PoseArm/1 -> IK/1, GraspPose/1, PoseErrCalc/2(Td)
  YawToBase/1 -> PoseWorld/1  "YawToBase"
  TfArmFromMap/1 -> ArmFrameEuler/1, PoseArm/1
  HeadingBack/1 -> YawToBase/2  "HeadingBack"

== system homeMobileManipulator/MobileManipulator/Manipulator/MotionPlanning/CandidateIK/Candidate_2 ==
  GraspPoint : Inport
  TfArmFromMap : Inport  Port=2
  IkGuess : Inport  Port=3
  IkWeights : Inport  Port=4
  ApproachEuler : Constant  Value=[cfg.plan.candidateYaw(2); cfg.plan.approachPitch; 0]
  ArmFrameEuler : robotcorelib/Coordinate Transformation Conversion  InputRepresentation=Homogeneous Transformation  InputEulerSequence=ZYX  ShowTrVecInputPort=off  OutputRepresentation=Euler Angles  OutputEulerSequence=ZYX  ShowTrVecOutputPort=off  SimulateUsing=Code generation
  HeadingBack : Gain  Gain=[-1 0 0; 0 0 0; 0 0 0]  Multiplication=Matrix(K*u)
  IK : robotmaniplib/Inverse Kinematics  RigidBodyTree=armIkTree  EndEffector=tcp_frame  ShowInfo=off  SolverName=BFGS Gradient Projection  EnforceJointLimits=on  AllowRandomRestarts=on  MaxIterations=cfg.plan.ikMaxIterations  MaxTime=cfg.plan.ikMaxTime  GradientTolerance=1e-7  SolutionTolerance=1e-6  StepTolerance=1e-14  ConstraintTolerance=1e-6  ErrorChangeTolerance=1e-12  UseErrorDamping=on  DampingBias=0.0025  RandomStream=mt19937ar with seed  Seed=cfg.plan.ikSeed  SimulateUsing=Code generation
  JJt : Product  Multiplication=Matrix(*)
  Jac : robotmaniplib/Get Jacobian  RigidBodyTree=armIkTree  EndEffector=tcp_frame  SimulateUsing=Code generation
  JacT : Math  Operator=transpose  SignedPower=on  RndMeth=Zero
  Manip : dspmtrx3/Reciprocal Condition
  PoseArm : Product  Multiplication=Matrix(*)
  PoseErrCalc : Subsystem  Description=Weighted twist between the achieved (Ta) and desired (Td) tool pose - the Inverse Kinematics block's PoseErrorNorm, rebuilt because its Info port cannot compile in this release. Blocks replace the former MATLAB Function (2026-10-14): inv(Ta)*Td, Coordinate Transformation Conversion to axis-angle and translation, weights in RST order (3 orientation, 3 position), 2-norm. Matched the function to 6.3e-9 worst case over 300 pose pairs, 2e-17 median.
  PoseWorld : robotcorelib/Coordinate Transformation Conversion  InputRepresentation=Euler Angles  InputEulerSequence=ZYX  ShowTrVecInputPort=on  OutputRepresentation=Homogeneous Transformation  OutputEulerSequence=ZYX  ShowTrVecOutputPort=off  SimulateUsing=Code generation
  TcpTf : robotmaniplib/Get Transform  RigidBodyTree=armIkTree  SourceBody=tcp_frame  TargetBody=arm_mount  SimulateUsing=Code generation
  YawToBase : Sum  Description=Yaw measured from the ARM base - see Candidate_1/YawToBase.
  Config : Outport
  PoseError : Outport  Port=2
  Manipulability : Outport  Port=3
  GraspPose : Outport  Port=4
  wires:
  Manip/1 -> Manipulability/1
  JJt/1 -> Manip/1  "JJt"
  PoseErrCalc/1(poseErrNorm) -> PoseError/1
  TcpTf/1 -> PoseErrCalc/1(Ta)
  IK/1 -> Jac/1, TcpTf/1, Config/1
  Jac/1 -> JacT/1, JJt/1
  IkGuess/1 -> IK/3
  PoseWorld/1 -> PoseArm/2
  YawToBase/1 -> PoseWorld/1  "YawToBase"
  ApproachEuler/1 -> YawToBase/1
  GraspPoint/1 -> PoseWorld/2
  JacT/1 -> JJt/2  "JacT"
  ArmFrameEuler/1 -> HeadingBack/1
  TfArmFromMap/1 -> ArmFrameEuler/1, PoseArm/1
  HeadingBack/1 -> YawToBase/2  "HeadingBack"
  PoseArm/1 -> PoseErrCalc/2(Td), GraspPose/1, IK/1
  IkWeights/1 -> IK/2, PoseErrCalc/3(w)

== system homeMobileManipulator/MobileManipulator/Manipulator/MotionPlanning/CandidateIK/Candidate_3 ==
  GraspPoint : Inport
  TfArmFromMap : Inport  Port=2
  IkGuess : Inport  Port=3
  IkWeights : Inport  Port=4
  ApproachEuler : Constant  Value=[cfg.plan.candidateYaw(3); cfg.plan.approachPitch; 0]
  ArmFrameEuler : robotcorelib/Coordinate Transformation Conversion  InputRepresentation=Homogeneous Transformation  InputEulerSequence=ZYX  ShowTrVecInputPort=off  OutputRepresentation=Euler Angles  OutputEulerSequence=ZYX  ShowTrVecOutputPort=off  SimulateUsing=Code generation
  HeadingBack : Gain  Gain=[-1 0 0; 0 0 0; 0 0 0]  Multiplication=Matrix(K*u)
  IK : robotmaniplib/Inverse Kinematics  RigidBodyTree=armIkTree  EndEffector=tcp_frame  ShowInfo=off  SolverName=BFGS Gradient Projection  EnforceJointLimits=on  AllowRandomRestarts=on  MaxIterations=cfg.plan.ikMaxIterations  MaxTime=cfg.plan.ikMaxTime  GradientTolerance=1e-7  SolutionTolerance=1e-6  StepTolerance=1e-14  ConstraintTolerance=1e-6  ErrorChangeTolerance=1e-12  UseErrorDamping=on  DampingBias=0.0025  RandomStream=mt19937ar with seed  Seed=cfg.plan.ikSeed  SimulateUsing=Code generation
  JJt : Product  Multiplication=Matrix(*)
  Jac : robotmaniplib/Get Jacobian  RigidBodyTree=armIkTree  EndEffector=tcp_frame  SimulateUsing=Code generation
  JacT : Math  Operator=transpose  SignedPower=on  RndMeth=Zero
  Manip : dspmtrx3/Reciprocal Condition
  PoseArm : Product  Multiplication=Matrix(*)
  PoseErrCalc : Subsystem  Description=Weighted twist between the achieved (Ta) and desired (Td) tool pose - the Inverse Kinematics block's PoseErrorNorm, rebuilt because its Info port cannot compile in this release. Blocks replace the former MATLAB Function (2026-10-14): inv(Ta)*Td, Coordinate Transformation Conversion to axis-angle and translation, weights in RST order (3 orientation, 3 position), 2-norm. Matched the function to 6.3e-9 worst case over 300 pose pairs, 2e-17 median.
  PoseWorld : robotcorelib/Coordinate Transformation Conversion  InputRepresentation=Euler Angles  InputEulerSequence=ZYX  ShowTrVecInputPort=on  OutputRepresentation=Homogeneous Transformation  OutputEulerSequence=ZYX  ShowTrVecOutputPort=off  SimulateUsing=Code generation
  TcpTf : robotmaniplib/Get Transform  RigidBodyTree=armIkTree  SourceBody=tcp_frame  TargetBody=arm_mount  SimulateUsing=Code generation
  YawToBase : Sum  Description=Yaw measured from the ARM base - see Candidate_1/YawToBase.
  Config : Outport
  PoseError : Outport  Port=2
  Manipulability : Outport  Port=3
  GraspPose : Outport  Port=4
  wires:
  Manip/1 -> Manipulability/1
  JJt/1 -> Manip/1  "JJt"
  JacT/1 -> JJt/2  "JacT"
  Jac/1 -> JacT/1, JJt/1
  TcpTf/1 -> PoseErrCalc/1(Ta)
  PoseErrCalc/1(poseErrNorm) -> PoseError/1
  IK/1 -> Jac/1, TcpTf/1, Config/1
  IkGuess/1 -> IK/3
  IkWeights/1 -> IK/2, PoseErrCalc/3(w)
  PoseWorld/1 -> PoseArm/2
  YawToBase/1 -> PoseWorld/1  "YawToBase"
  HeadingBack/1 -> YawToBase/2  "HeadingBack"
  GraspPoint/1 -> PoseWorld/2
  ApproachEuler/1 -> YawToBase/1
  ArmFrameEuler/1 -> HeadingBack/1
  PoseArm/1 -> GraspPose/1, IK/1, PoseErrCalc/2(Td)
  TfArmFromMap/1 -> ArmFrameEuler/1, PoseArm/1

== system homeMobileManipulator/MobileManipulator/MobileBase/PathFollowing/TrackingError/BodyRotation ==
  BasePose : Inport
  PlanarBlock : Selector  NumberOfDimensions=2  InputPortWidth=3  IndexOptions=Index vector (dialog),Index vector (dialog)  Indices=[1 2],[1 2]  OutputSizes=1
  WorldToBody : Math  Operator=transpose
  YawSelect : Gain  Gain=[0 0 1; 0 0 0; 0 0 0]  Multiplication=Matrix(K*u)
  YawToRotation : robotcorelib/Coordinate Transformation Conversion  InputRepresentation=Euler Angles  InputEulerSequence=ZYX  ShowTrVecInputPort=off  OutputRepresentation=Rotation Matrix  OutputEulerSequence=ZYX  ShowTrVecOutputPort=off  SimulateUsing=Code generation
  RotBodyFromWorld : Outport
  wires:
  PlanarBlock/1 -> RotBodyFromWorld/1
  WorldToBody/1 -> PlanarBlock/1  "WorldToBody"
  YawToRotation/1 -> WorldToBody/1
  YawSelect/1 -> YawToRotation/1  "YawSelect"
  BasePose/1 -> YawSelect/1

== system homeMobileManipulator/MobileManipulator/Plant/CameraRig/WristCamera/WristMountPose ==
  RobotConfig : Inport
  RelRotationRow : Reshape  OutputDimensionality=Row vector (2-D)
  RelTranslationRow : Reshape  OutputDimensionality=Row vector (2-D)
  RotToUnreal : Gain  Gain=[0 0 -1; 0 -1 0; 1 0 0]  Multiplication=Matrix(K*u)
  WristCamPose : robotmaniplib/Get Transform  RigidBodyTree=robot  SourceBody=wrist_cam  TargetBody=map  SimulateUsing=Code generation
  WristCamToEuler : robotcorelib/Coordinate Transformation Conversion  InputRepresentation=Homogeneous Transformation  InputEulerSequence=ZYX  ShowTrVecInputPort=on  OutputRepresentation=Euler Angles  OutputEulerSequence=ZYX  ShowTrVecOutputPort=on  SimulateUsing=Code generation
  RelTranslation : Outport
  RelRotation : Outport  Port=2
  wires:
  RelRotationRow/1 -> RelRotation/1
  RotToUnreal/1 -> RelRotationRow/1  "RotToUnreal"
  WristCamToEuler/1 -> RotToUnreal/1
  RelTranslationRow/1 -> RelTranslation/1
  WristCamPose/1 -> WristCamToEuler/1  "WristCamInParent"
  RobotConfig/1 -> WristCamPose/1
  WristCamToEuler/2 -> RelTranslationRow/1

== system homeMobileManipulator/MobileManipulator/Manipulator/MotionPlanning/CandidateIK/Candidate_1/PoseErrCalc ==
  Ta : Inport
  Td : Inport  Port=2
  w : Inport  Port=3
  Angle : Selector  InputPortWidth=4  IndexOptions=Index vector (dialog)  Indices=4  OutputSizes=1
  Axis : Selector  InputPortWidth=4  IndexOptions=Index vector (dialog)  Indices=1:3  OutputSizes=1
  ErrorTform : Product  Inputs=/*  Multiplication=Matrix(*)
  Norm : Sqrt
  OrientWeights : Selector  InputPortWidth=6  IndexOptions=Index vector (dialog)  Indices=1:3  OutputSizes=1
  PosWeights : Selector  InputPortWidth=6  IndexOptions=Index vector (dialog)  Indices=4:6  OutputSizes=1
  RotationVector : Product  Inputs=**
  SumSquares : DotProduct  OutDataTypeStr=Inherit: Inherit via internal rule
  ToAxisAngle : robotcorelib/Coordinate Transformation Conversion  InputRepresentation=Homogeneous Transformation  InputEulerSequence=ZYX  ShowTrVecInputPort=on  OutputRepresentation=Axis-Angle  OutputEulerSequence=ZYX  ShowTrVecOutputPort=on  SimulateUsing=Code generation
  WeightOrient : Product  Inputs=**
  WeightPos : Product  Inputs=**
  WeightedTwist : Concatenate
  poseErrNorm : Outport
  wires:
  SumSquares/1 -> Norm/1  "SumSquares"
  WeightedTwist/1 -> SumSquares/1, SumSquares/2
  WeightPos/1 -> WeightedTwist/2  "WeightPos"
  WeightOrient/1 -> WeightedTwist/1  "WeightOrient"
  PosWeights/1 -> WeightPos/2
  OrientWeights/1 -> WeightOrient/2
  RotationVector/1 -> WeightOrient/1  "RotationVector"
  Axis/1 -> RotationVector/1
  Norm/1 -> poseErrNorm/1
  ToAxisAngle/2 -> WeightPos/1
  ToAxisAngle/1 -> Axis/1, Angle/1
  Angle/1 -> RotationVector/2
  Td/1 -> ErrorTform/2
  ErrorTform/1 -> ToAxisAngle/1  "ErrorTform"
  Ta/1 -> ErrorTform/1
  w/1 -> OrientWeights/1, PosWeights/1
